simulink model "sm_robot_run_03_leg_inverse_dyn"  (R2025a)
settings: Solver=ode15s  StartTime=0.0  StopTime=max(TimeValues)  MaxStep=1e-3  RelTol=1e-3  AbsTol=1e-4  EnableMultiTasking=on
InitFcn:
  | r2d=180/pi;
  | if (~exist('TimeValues'))
  |   sm_robot_run_4legs_param_def_load(bdroot)
  | end
values from neighbouring files (symbols this model uses):
  N = 100    [Extr_Data_Cam_Roller_Curve.m]
  s = sin(q)    [Extr_Data_Cam_Roller_Curve.m]
undefined symbols (not defined in the file or in its folder): l1, l2, m1, m2, T_cg, th1, th2
libraries: nesl_utility x8, sm_lib x6
CloseFcn:
  | try,close(h1_sm_robot_run_03_leg_inverse_dyn),end
  | clear h1_sm_robot_run_03_leg_inverse_dyn
  | 
  | clear simlog_sm_robot_run_03_leg_inverse_dyn
  | clear logsout_sm_robot_run_03_leg_inverse_dyn
Description:
  | Robot Leg Inverse Dynamics
  | 
  | Copyright 2012-2025 The MathWorks, Inc.
settings Model: Creator=rhyde  LastModifiedBy=smiller
settings SolverCC: AutoScaleAbsTol=off  MaxConsecutiveZCs=10000  AlgebraicLoopSolver=TrustRegion
settings DataIOCC: LimitDataPoints=on  MaxDataPoints=10000  SaveFinalState=on  SaveFormat=Array  SaveState=on  ReturnWorkspaceOutputs=off  SignalLoggingName=logsout_sm_robot_run_03_leg_inverse_dyn  OutputTimes=[0:0.01:max(TimeValues)]
settings OptimizationCC: ReuseModelBlockBuffer=off  ExpressionDepthLimit=2147483647.0  InitFltsAndDblsToZero=on  LifeSpan=inf
settings DebuggingCC: SaveWithParameterizedLinksMsg=none  UnderspecifiedInitializationDetection=Classic  MergeDetectMultiDrivingBlocksExec=none  SignalResolutionControl=TryResolveAllWithWarning  SolverPrmCheckMsg=warning  MultiTaskDSMMsg=warning  MultiTaskCondExecSysMsg=none  FcnCallInpInsideContextMsg=warning  UnconnectedInputMsg=warning  UnconnectedOutputMsg=warning  UnconnectedLineMsg=warning  StateNameClashWarn=warning  PregeneratedLibrarySubsystemCodeDiagnostic=none  SFUnexpectedBacktrackingDiag=warning  SFNoUnconditionalDefaultTransitionDiag=warning  SFExecutionAtInitializationDiag=none  ArithmeticOperatorsInVariantConditions=warning
settings HardwareCC: ProdBitPerPointer=32.0  ProdBitPerSizeT=32.0  ProdBitPerPtrDiffT=32.0  ProdLargestAtomicFloat=None  ProdIntDivRoundTo=Undefined  ProdEndianess=Unspecified  ProdWordSize=32.0  ProdHWDeviceType=32-bit Generic
settings ModelReferenceCC: EnableRefExpFcnMdlSchedulingChecks=on  PropagateSignalLabelsOutOfModel=off
settings SFSimCC: SimUseLocalCustomCode=off  CustomCodeUndefinedFunction=UseInterfaceOnly
settings RTWCC: RTWUseLocalCustomCode=off  GPUComputeCapability=3.5  DLArmComputeVersion=19.05
settings CodeAppCC: StateflowObjectComments=on
settings GRTTargetCC: TargetFcnLib=ansi_tfl_tmw.mat  TargetLangStandard=C89/C90 (ANSI)  CombineOutputUpdateFcns=off  GRTInterface=on
settings ConfigComp: CovMetricSettings=dw  CovSaveCumulativeToWorkspaceVar=on  CovSaveSingleToWorkspaceVar=on  CovExternalEMLEnable=off
settings SimscapeCC: SimscapeNormalizeSystem=off  SimscapeLogType=all  SimscapeLogSimulationStatistics=on  SimscapeLogName=simlog_sm_robot_run_03_leg_inverse_dyn  SimscapeLogDataHistory=10000.0
settings ConfigurationSet: Description=SimMechanics 2G
settings ExplorerConfigSet: InternalSimMechanicsExplorerSettings="<ExplorerConfiguration><canonicalview>default</canonicalview><AnimationSetting><BasePlaybackSpeed>1.0</BasePlaybackSpeed><PlaybackSpeedFactor>1.0</PlaybackSpeedFactor></AnimationSetting><TilePanel><TileInfo><Tiles Columns=\"1\" Count=\"1\" Rows=\"1\"><Column Left=\"2\" Weight=\"1\"/><Column Left=\"697\"/><Row Top=\"2\" Weight=\"1\"/><Row Top=\"430\"/><Tile Height=\"1\" Width=\"1\" X=\"0\" Y=\"0\"/></Tiles></TileInfo><SceneInfo><SceneViewer><BGColor><R>1</R><G>1</G><B>1</B></BGColor><Camera><DoPerspective>off</DoPerspective><Position><X>0.12448516488075256</X><Y>-0.4990077018737793</Y><Z>1.0000000000000004</Z></Position><Center><X>0.12448516488075256</X><Y>-0.4990077018737793</Y><Z>4.4408920985006262e-16</Z></Center><Up><X>0</X><Y>1</Y><Z>-0</Z></Up><ViewLimDist>1</ViewLimDist><YLim>0.52676334857940676</YLim><XLim>0.86243354922547266</XLim></Camera></SceneViewer></SceneInfo></TilePanel><MechEditorPanel><Cameras/><GfxPanelCameraMap/><VideoCreator><PlaybackSpeedRatio>1.0</PlaybackSpeedRatio><FrameRate>30</FrameRate><VideoFormat>Motion JPEG AVI</VideoFormat><FrameSize>auto</FrameSize></VideoCreator></MechEditorPanel></ExplorerConfiguration>"

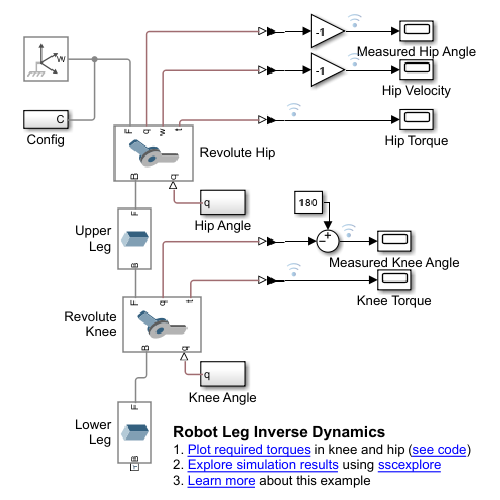
[thumbnail: Simulink's stored preview of the top-level diagram]
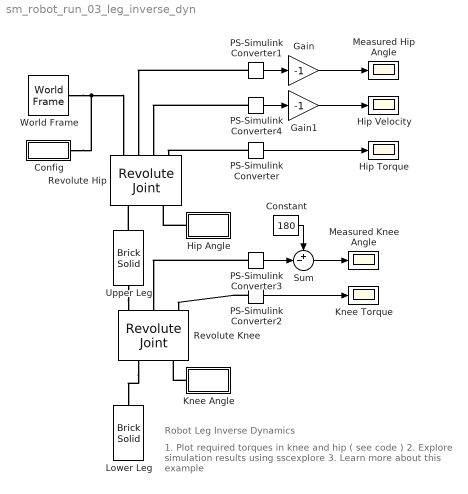
== system sm_robot_run_03_leg_inverse_dyn ==
  note: Robot Leg Inverse Dynamics
  note: 1. Plot required torques in knee and hip ( see code )
      | 2. Explore simulation results using sscexplore
      | 3. Learn more about this example
  Config : Subsystem
  Constant : Constant  Value=180
  Gain : Gain  Gain=-1
  Gain1 : Gain  Gain=-1
  Hip Angle : Subsystem
  Hip Torque : Scope
      settings: DataLoggingVariableName=hip_torque
  Hip Velocity : Scope
      settings: TimeSpan=1.5  ActiveDisplayYMinimum=-173.79097  ActiveDisplayYMaximum=222.43934  DataLoggingVariableName=HipVel
  Knee Angle : Subsystem
  Knee Torque : Scope
      settings: TimeSpan=1.488  ActiveDisplayYMinimum=-121.47298  ActiveDisplayYMaximum=113.41881  DataLoggingVariableName=knee_torque
  Lower Leg : sm_lib/Body Elements/Brick Solid  BrickDimensions=[0.1 1 0.1]*l2  BrickDimensionsUnits=m  ExportEntireGeometry=off  InertiaType=Custom  BasedOnType=Density  Density=1000  DensityUnits=kg/m^3  Mass=m2*l2  MassUnits=kg  CenterOfMass=[0 0 0]  CenterOfMassUnits=m  MomentsOfInertia=[1 1 1]*(1/12)*m2*l2*l2^2  MomentsOfInertiaUnits=kg*m^2  ProductsOfInertia=[1 1 1]*0  ProductsOfInertiaUnits=kg*m^2  GraphicType=FromGeometry  MarkerShape=Sphere  MarkerSize=10  GraphicVisPropType=SimpleVisualProperties  GraphicDiffuseColor=[0.5 0.5 0.5]  GraphicOpacity=1.0  GraphicSpecularColor=[0.5 0.5 0.5 1.0]  GraphicAmbientColor=[0.15 0.15 0.15 1.0]  GraphicEmissiveColor=[0.0 0.0 0.0 1.0]  GraphicShininess=75  DoExposeReferenceFrame=off  SerializedFrames=<Frames><Frame><Id>Frame1</Id><Value><Name>B</Name><Origin><Source>GeometricFeature</Source><FeatureName>-y surface</FeatureName></Origin><PrimaryAxis><DefinedDirection>+Z</DefinedDirection><Source>ReferenceFrame</Source><SourceDirection>+Z</SourceDirection><FeatureName></FeatureName></PrimaryAxis><SecondaryAxis><DefinedDirection>+X</DefinedDirection><Source>ReferenceFrame</Source><SourceDirection>+X</SourceDirection><FeatureName></FeatureName></SecondaryAxis></Value></Frame><Frame><Id>Frame2</Id><Value><Name>F</Name><Origin><Source>GeometricFeature</Source><FeatureName>+y surface</FeatureName></Origin><PrimaryAxis><DefinedDirection>+Z</DefinedDirection><Source>ReferenceFrame</Source><SourceDirection>+Z</SourceDirection><FeatureName></FeatureName></PrimaryAxis><SecondaryAxis><DefinedDirection>+X</DefinedDirection><Source>ReferenceFrame</Source><SourceDirection>+X</SourceDirection><FeatureName></FeatureName></SecondaryAxis></Value></Frame></Frames>
  Measured Hip Angle : Scope
      settings: TimeSpan=1.5  ActiveDisplayYMinimum=-2.42306  ActiveDisplayYMaximum=52.42306  DataLoggingVariableName=Hip
  Measured Knee Angle : Scope
      settings: TimeSpan=1.488  ActiveDisplayYMinimum=71.22313  ActiveDisplayYMaximum=136.53076  DataLoggingVariableName=Knee
  PS-Simulink Converter : nesl_utility/PS-Simulink Converter  PhysicalDomain=network_engine_domain  SubClassName=ps_output  LeftPortType=input  RightPortType=output  PseudoPeriodic=off  Frequencies=[]  VectorFormat=1-D array  Unit=1  AffineConversion=off
  PS-Simulink Converter1 : nesl_utility/PS-Simulink Converter  PhysicalDomain=network_engine_domain  SubClassName=ps_output  LeftPortType=input  RightPortType=output  PseudoPeriodic=off  Frequencies=[]  VectorFormat=1-D array  Unit=deg  AffineConversion=off
  PS-Simulink Converter2 : nesl_utility/PS-Simulink Converter  PhysicalDomain=network_engine_domain  SubClassName=ps_output  LeftPortType=input  RightPortType=output  PseudoPeriodic=off  Frequencies=[]  VectorFormat=1-D array  Unit=1  AffineConversion=off
  PS-Simulink Converter3 : nesl_utility/PS-Simulink Converter  PhysicalDomain=network_engine_domain  SubClassName=ps_output  LeftPortType=input  RightPortType=output  PseudoPeriodic=off  Frequencies=[]  VectorFormat=1-D array  Unit=deg  AffineConversion=off
  PS-Simulink Converter4 : nesl_utility/PS-Simulink Converter  PhysicalDomain=network_engine_domain  SubClassName=ps_output  LeftPortType=input  RightPortType=output  PseudoPeriodic=off  Frequencies=[]  VectorFormat=1-D array  Unit=deg/s  AffineConversion=off
  Revolute Knee : sm_lib/Joints/Revolute Joint  JointMode=Normal  CompositeWrenchDir=FollowerOnBase  CompositeWrenchFrame=BaseFrame  SenseConstraintForce=off  SenseConstraintTorque=off  SenseTotalForce=off  SenseTotalTorque=off  PositionTargetSpecify=on  PositionTargetPriority=High  PositionTargetValue=-th2+pi  PositionTargetValueUnits=rad  VelocityTargetSpecify=off  VelocityTargetPriority=High  VelocityTargetValue=0  VelocityTargetValueUnits=rad/s  EquilibriumPosition=0  EquilibriumPositionUnits=deg  SpringStiffness=0  SpringStiffnessUnits=N*m/deg  DampingCoefficient=0  DampingCoefficientUnits=N*m/(deg/s)  LowerLimitSpecify=off  LowerLimitBound=-90  LowerLimitBoundUnits=deg  LowerLimitStiffness=1e4  LowerLimitStiffnessUnits=N*m/deg  LowerLimitDamping=10  LowerLimitDampingUnits=N*m/(deg/s)  LowerLimitTransitionRegionWidth=0.1  LowerLimitTransitionRegionWidthUnits=deg  UpperLimitSpecify=off  UpperLimitBound=90  UpperLimitBoundUnits=deg  UpperLimitStiffness=1e4  UpperLimitStiffnessUnits=N*m/deg  UpperLimitDamping=10  UpperLimitDampingUnits=N*m/(deg/s)  UpperLimitTransitionRegionWidth=0.1  UpperLimitTransitionRegionWidthUnits=deg  TorqueActuationMode=ComputedTorque  MotionActuationMode=InputMotion  SensePosition=on  SenseVelocity=off  SenseAcceleration=off  SenseTorqueForce=on  SenseLowerLimitTorqueForce=off  SenseUpperLimitTorqueForce=off
  Revolute Hip : sm_lib/Joints/Revolute Joint  JointMode=Normal  CompositeWrenchDir=FollowerOnBase  CompositeWrenchFrame=BaseFrame  SenseConstraintForce=off  SenseConstraintTorque=off  SenseTotalForce=off  SenseTotalTorque=off  PositionTargetSpecify=on  PositionTargetPriority=High  PositionTargetValue=-th1  PositionTargetValueUnits=rad  VelocityTargetSpecify=off  VelocityTargetPriority=High  VelocityTargetValue=0  VelocityTargetValueUnits=rad/s  EquilibriumPosition=0  EquilibriumPositionUnits=deg  SpringStiffness=0  SpringStiffnessUnits=N*m/deg  DampingCoefficient=0  DampingCoefficientUnits=N*m/(deg/s)  LowerLimitSpecify=off  LowerLimitBound=-90  LowerLimitBoundUnits=deg  LowerLimitStiffness=1e4  LowerLimitStiffnessUnits=N*m/deg  LowerLimitDamping=10  LowerLimitDampingUnits=N*m/(deg/s)  LowerLimitTransitionRegionWidth=0.1  LowerLimitTransitionRegionWidthUnits=deg  UpperLimitSpecify=off  UpperLimitBound=90  UpperLimitBoundUnits=deg  UpperLimitStiffness=1e4  UpperLimitStiffnessUnits=N*m/deg  UpperLimitDamping=10  UpperLimitDampingUnits=N*m/(deg/s)  UpperLimitTransitionRegionWidth=0.1  UpperLimitTransitionRegionWidthUnits=deg  TorqueActuationMode=ComputedTorque  MotionActuationMode=InputMotion  SensePosition=on  SenseVelocity=on  SenseAcceleration=off  SenseTorqueForce=on  SenseLowerLimitTorqueForce=off  SenseUpperLimitTorqueForce=off
  Sum : Sum  Inputs=+-|
  Upper Leg : sm_lib/Body Elements/Brick Solid  BrickDimensions=[0.1 1 0.1]*l1  BrickDimensionsUnits=m  ExportEntireGeometry=off  InertiaType=Custom  BasedOnType=Density  Density=1000  DensityUnits=kg/m^3  Mass=m1*l1  MassUnits=kg  CenterOfMass=[0 0 0]  CenterOfMassUnits=m  MomentsOfInertia=[1 1 1]*(1/12)*m1*l1*l1^2  MomentsOfInertiaUnits=kg*m^2  ProductsOfInertia=[1 1 1]*0  ProductsOfInertiaUnits=kg*m^2  GraphicType=FromGeometry  MarkerShape=Sphere  MarkerSize=10  GraphicVisPropType=SimpleVisualProperties  GraphicDiffuseColor=[0.5 0.5 0.5]  GraphicOpacity=1.0  GraphicSpecularColor=[0.5 0.5 0.5 1.0]  GraphicAmbientColor=[0.15 0.15 0.15 1.0]  GraphicEmissiveColor=[0.0 0.0 0.0 1.0]  GraphicShininess=75  DoExposeReferenceFrame=off  SerializedFrames=<Frames><Frame><Id>Frame1</Id><Value><Name>B</Name><Origin><Source>GeometricFeature</Source><FeatureName>-y surface</FeatureName></Origin><PrimaryAxis><DefinedDirection>+Z</DefinedDirection><Source>ReferenceFrame</Source><SourceDirection>+Z</SourceDirection><FeatureName></FeatureName></PrimaryAxis><SecondaryAxis><DefinedDirection>+X</DefinedDirection><Source>ReferenceFrame</Source><SourceDirection>+X</SourceDirection><FeatureName></FeatureName></SecondaryAxis></Value></Frame><Frame><Id>Frame2</Id><Value><Name>F</Name><Origin><Source>GeometricFeature</Source><FeatureName>+y surface</FeatureName></Origin><PrimaryAxis><DefinedDirection>+Z</DefinedDirection><Source>ReferenceFrame</Source><SourceDirection>+Z</SourceDirection><FeatureName></FeatureName></PrimaryAxis><SecondaryAxis><DefinedDirection>+X</DefinedDirection><Source>ReferenceFrame</Source><SourceDirection>+X</SourceDirection><FeatureName></FeatureName></SecondaryAxis></Value></Frame></Frames>
  World Frame : sm_lib/Frames and Transforms/World Frame
  wires:
  PS-Simulink Converter3/1 -> Sum/2
  PS-Simulink Converter2/1 -> Knee Torque/1
  PS-Simulink Converter/1 -> Hip Torque/1
  PS-Simulink Converter1/1 -> Gain/1
  Gain/1 -> Measured Hip Angle/1
  Constant/1 -> Sum/1
  Sum/1 -> Measured Knee Angle/1
  Gain1/1 -> Hip Velocity/1
  PS-Simulink Converter4/1 -> Gain1/1
  connections:
  Revolute Knee/LConn1 -- Lower Leg/RConn1
  Upper Leg/LConn1 -- Revolute Knee/RConn1
  Upper Leg/RConn1 -- Revolute Hip/LConn1
  World Frame/RConn1 -- Revolute Hip/RConn1 -- Config/RConn1
  PS-Simulink Converter/LConn1 -- Revolute Hip/RConn4
  PS-Simulink Converter1/LConn1 -- Revolute Hip/RConn2
  PS-Simulink Converter3/LConn1 -- Revolute Knee/RConn2
  PS-Simulink Converter2/LConn1 -- Revolute Knee/RConn3
  Hip Angle/RConn1 -- Revolute Hip/LConn2
  Knee Angle/RConn1 -- Revolute Knee/LConn2
  PS-Simulink Converter4/LConn1 -- Revolute Hip/RConn3

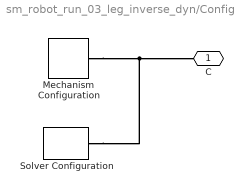
== system sm_robot_run_03_leg_inverse_dyn/Config ==
  Mechanism Configuration : sm_lib/Utilities/Mechanism Configuration  UniformGravity=Constant  GravityVector=[0 -9.81 0]  GravityVectorUnits=m/s^2  LinearizationDelta=0.001  JointModeTransitionNonlinearIterations=2
  Solver Configuration : nesl_utility/Solver Configuration  PhysicalDomain=network_engine_domain  SubClassName=solver  LeftPortType=input  RightPortType=generic  Tones=[]  Harmonics=[]  SimulateNoise=off  Profile=off  UseLocalSampling=off  EnableSwitchedLinearOptims=on  FrequencyDomain=off  UseCCode=off  RelTol=0.001  AbsTol=1e-06  MinStep=1e-09  ToWorkspace=off  RevertToSquareIcSolve=off  NumHomotopyIterations=100  PhasorMode=off  PhasorModeNumHarmonics=1  ConsistencySolver=NEWTON_FTOL  IndexReductionMethod=DerivativeReplacement  DoDC=off  ResidualTolerance=1e-09  ConsistencyTolSource=GLOBAL  ConsistencyAbsTol=0.001  ConsistencyRelTol=0.001  ConsistencyTolFactor=0.001  UseLocalSolver=off  LocalSolverChoice=NE_BACKWARD_EULER_ADVANCER  ResolveIndetEquations=on  FunctionEvalNumThread=1  LocalSolverSampleTime=0.001  DoFixedCost=off  MaxNonlinIter=3  MaxModeIter=2  ComputeImpulses=off  ImpulseIterations=2  LinearAlgebra=Sparse  LinearAlgebraNumThread=0  EquationFormulation=NE_TIME_EF  DelaysMemoryBudget=1024  AutomaticFiltering=on  FilteringTimeConstant=0.001  PartitionStorageMethod=AS_NEEDED  PartitionMemoryBudget=1024  PartitionMethod=FAST  MultibodyUseLocalSolver=off  MultibodyLocalSolverChoice=ODE1  MultibodyLocalSolverSampleTime=0.001
  C : PMIOPort  Side=Right
  connections:
  Mechanism Configuration/RConn1 -- C/RConn1 -- Solver Configuration/RConn1

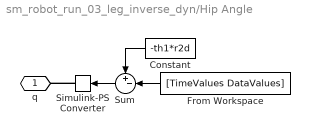
== system sm_robot_run_03_leg_inverse_dyn/Hip Angle ==
  Constant : Constant  Value=-th1*r2d
  From Workspace : FromWorkspace  VariableName=[TimeValues DataValues]
  Simulink-PS Converter : nesl_utility/Simulink-PS Converter  PhysicalDomain=network_engine_domain  SubClassName=ps_input  LeftPortType=input  RightPortType=output  PseudoPeriodic=off  Frequencies=[]  NoiseDistribution=none  NoiseParameters=[]  Unit=deg  AffineConversion=off  FilteringAndDerivatives=filter  SimscapeFilterOrder=2  InputFilterTimeConstant=0.005  UdotUserProvided=2
  Sum : Sum  Inputs=+-|
  q : PMIOPort  Side=Right
  wires:
  Constant/1 -> Sum/1
  Sum/1 -> Simulink-PS Converter/1
  From Workspace/1 -> Sum/2
  connections:
  Simulink-PS Converter/RConn1 -- q/RConn1

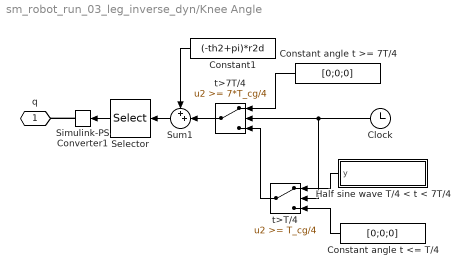
== system sm_robot_run_03_leg_inverse_dyn/Knee Angle ==
  Clock : Clock
  Constant angle t <= T/4 : Constant  Value=[0;0;0]
  Constant angle t >= 7T/4 : Constant  Value=[0;0;0]
  Constant1 : Constant  Value=(-th2+pi)*r2d
  Half sine wave T/4 < t < 7T/4 : Subsystem
  Selector : Selector  InputPortWidth=3  IndexOptions=Index vector (dialog)  Indices=1  OutputSizes=1
  Simulink-PS Converter1 : nesl_utility/Simulink-PS Converter  PhysicalDomain=network_engine_domain  SubClassName=ps_input  LeftPortType=input  RightPortType=output  PseudoPeriodic=off  Frequencies=[]  NoiseDistribution=none  NoiseParameters=[]  Unit=deg  AffineConversion=off  FilteringAndDerivatives=filter  SimscapeFilterOrder=2  InputFilterTimeConstant=0.005  UdotUserProvided=2
  Sum1 : Sum  Inputs=++|
  t>7T/4 : Switch  Threshold=7*T_cg/4  SaturateOnIntegerOverflow=off  InputSameDT=off
  t>T/4 : Switch  Threshold=T_cg/4  SaturateOnIntegerOverflow=off  InputSameDT=off
  q : PMIOPort  Side=Right
  wires:
  Sum1/1 -> Selector/1
  Selector/1 -> Simulink-PS Converter1/1
  Constant1/1 -> Sum1/1
  Half sine wave T/4 < t < 7T/4/1(y) -> t>T/4/1
  Constant angle t <= T/4/1 -> t>T/4/3
  t>T/4/1 -> t>7T/4/3
  Clock/1 -> t>T/4/2, t>7T/4/2
  Constant angle t >= 7T/4/1 -> t>7T/4/1
  t>7T/4/1 -> Sum1/2
  connections:
  Simulink-PS Converter1/RConn1 -- q/RConn1

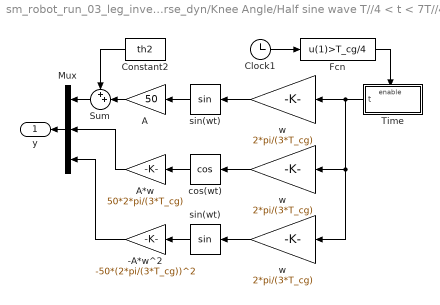
== system sm_robot_run_03_leg_inverse_dyn/Knee Angle/Half sine wave T//4 < t < 7T//4 ==
  -A*w^2 : Gain  Gain=-50*(2*pi/(3*T_cg))^2
  A : Gain  Gain=50
  A*w : Gain  Gain=50*2*pi/(3*T_cg)
  Clock1 : Clock
  Constant2 : Constant  Value=th2
  Fcn : Fcn  Expr=u(1)>T_cg/4
  Mux : Mux  Inputs=3
  Sum : Sum  Inputs=++|
  Time : Subsystem  TreatAsAtomicUnit=on
  cos(wt) : Trigonometry  Operator=cos
  sin(wt) : Trigonometry
  "sin(wt) " : Trigonometry
  w : Gain  Gain=2*pi/(3*T_cg)
  "w " : Gain  Gain=2*pi/(3*T_cg)
  "w  " : Gain  Gain=2*pi/(3*T_cg)
  y : Outport  VectorParamsAs1DForOutWhenUnconnected=off
  wires:
  Sum/1 -> Mux/1
  Constant2/1 -> Sum/1
  A*w/1 -> Mux/2
  Fcn/1 -> Time/Enable
  Clock1/1 -> Fcn/1
  A/1 -> Sum/2
  sin(wt)/1 -> A/1
  w/1 -> sin(wt)/1
  Time/1(t) -> w/1, "w "/1, "w  "/1
  cos(wt)/1 -> A*w/1
  "w "/1 -> cos(wt)/1
  "sin(wt) "/1 -> -A*w^2/1
  "w  "/1 -> "sin(wt) "/1
  -A*w^2/1 -> Mux/3
  Mux/1 -> y/1

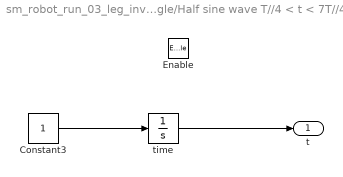
== system sm_robot_run_03_leg_inverse_dyn/Knee Angle/Half sine wave T//4 < t < 7T//4/Time ==
  Enable : EnablePort
  Constant3 : Constant
  time : Integrator
  t : Outport  InitialOutput=0  VectorParamsAs1DForOutWhenUnconnected=off
  wires:
  Constant3/1 -> time/1
  time/1 -> t/1
